simulink model "pendulum_sim_solver_test_block"  (R2016b)
settings: Solver=VariableStepAuto  StartTime=0.0  StopTime=10.0  RelTol=1e-3
libraries: simulink x1
settings Model: Creator=oj  LastModifiedBy=oj
settings DataIOCC: ReturnWorkspaceOutputs=on
settings DebuggingCC: UnconnectedInputMsg=none  UnconnectedOutputMsg=none  UnconnectedLineMsg=none
settings ModelReferenceCC: EnableRefExpFcnMdlSchedulingChecks=off
settings SFSimCC: SimUseLocalCustomCode=on
settings RTWCC: RTWUseLocalCustomCode=on

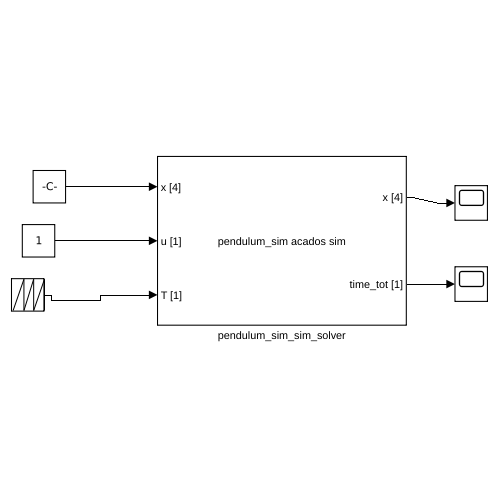
[thumbnail: Simulink's stored preview of the top-level diagram]
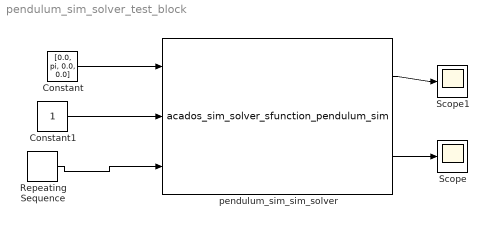
== system pendulum_sim_solver_test_block ==
  Constant : Constant  Value=[0.0, pi, 0.0, 0.0]
  Constant1 : Constant
  Repeating Sequence : simulink/Sources/Repeating Sequence  rep_seq_t=[0 2]  rep_seq_y=[0 2]
  Scope : Scope
  Scope1 : Scope
  pendulum_sim_sim_solver : S-Function  FunctionName=acados_sim_solver_sfunction_pendulum_sim  SFunctionDeploymentMode=off  EnableBusSupport=off
      mask Display:
      | port_label('input', 1, 'x [4]')
      | port_label('input', 2, 'u [1]')
      | port_label('input', 3, 'T [1]')
      | port_label('output', 1, 'x [4]')
      | port_label('output', 2, 'time_tot [1]')
      | disp('pendulum_sim acados sim')
  wires:
  pendulum_sim_sim_solver/2 -> Scope/1
  Constant/1 -> pendulum_sim_sim_solver/1
  Constant1/1 -> pendulum_sim_sim_solver/2
  pendulum_sim_sim_solver/1 -> Scope1/1
  Repeating Sequence/1 -> pendulum_sim_sim_solver/3
